simulink model "cart_pendulum_lqr_sim"  (R2025b)
settings: Solver=ode45  StartTime=0.0  StopTime=10.0  MaxStep=0.01  RelTol=1e-7  AbsTol=1e-9
values from neighbouring files (symbols this model uses):
  Fmax = 10    [cart_pendulum_lqr.m]
  K = newK    [cart_pendulum_application.m]    (also in cart_pendulum_lqr.m = lqr(A, B, Q, R))
  z0 = [0; 0; deg2rad(10); 0]    [cart_pendulum_lqr.m]
undefined symbols (not defined in the file or in its folder): p
settings Model: Creator=BATU  LastModifiedBy=BATU

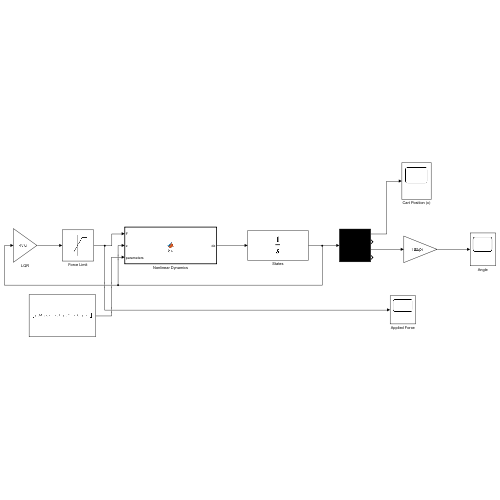
[thumbnail: Simulink's stored preview of the top-level diagram]
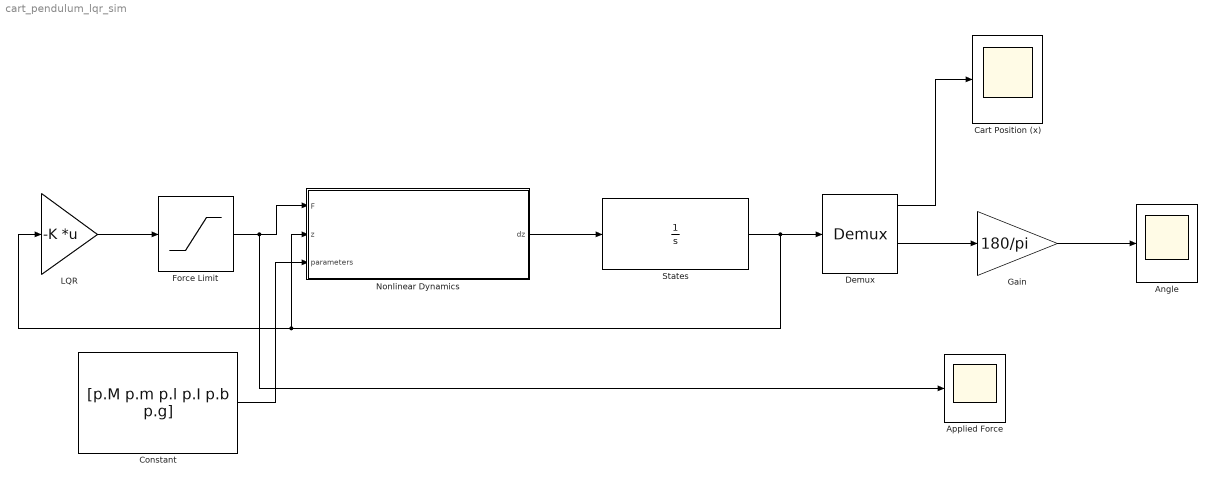
== system cart_pendulum_lqr_sim ==
  Angle : Scope
      settings: ActiveDisplayYMinimum=-5.1100864089155191  ActiveDisplayYMaximum=11.678898489879503
  Applied Force : Scope
      settings: ActiveDisplayYMinimum=-11.484305579852068  ActiveDisplayYMaximum=3.3587502186686171  DataLoggingVariableName=ScopeData2
  Cart Position (x) : Scope
      settings: ActiveDisplayYMinimum=-0.14782496214198251  ActiveDisplayYMaximum=0.016502017656709497
  Constant : Constant  Value=[p.M p.m p.l p.I p.b p.g]
  Demux : Demux
  Force Limit : Saturate  UpperLimit=Fmax  LowerLimit=-Fmax
  Gain : Gain  Gain=180/pi
  LQR : Gain  Gain=-K  Multiplication=Matrix(K*u)
  Nonlinear Dynamics : MATLAB Function  TreatAsAtomicUnit=on
  States : Integrator  InitialCondition=z0
  wires:
  LQR/1 -> Force Limit/1
  Force Limit/1 -> Applied Force/1, Nonlinear Dynamics/1(F)
  Nonlinear Dynamics/1(dz) -> States/1
  States/1 -> Demux/1, Nonlinear Dynamics/2(z), LQR/1
  Constant/1 -> Nonlinear Dynamics/3(parameters)
  Demux/1 -> Cart Position (x)/1
  Gain/1 -> Angle/1
  Demux/3 -> Gain/1

== matlab function cart_pendulum_lqr_sim/Nonlinear Dynamics ==
  data: F input; dz output; z input; parameters input
function dz = fcn(F, z, parameters)
% States: [x; velocity; theta; angular velocity]

M = parameters(1);
m = parameters(2);
l = parameters(3);
I = parameters(4);
b = parameters(5);
g = parameters(6);

v     = z(2);
theta = z(3);
omega = z(4);

J = I + m*l^2;
h = m*l;

H = [M + m,        -h*cos(theta);
     -h*cos(theta), J];

rhs = [F - b*v - h*sin(theta)*omega^2;
       h*g*sin(theta)];

acceleration = H \ rhs;

dz = [v;
      acceleration(1);
      omega;
      acceleration(2)];
end
